simulink model "bins_model"  (Simulink 7.9)
settings: Solver=ode23  StartTime=0.0  StopTime=12  MaxStep=0.01  RelTol=1e-6
settings Model: Creator=S  LastModifiedBy=S
settings SolverCC: SolverResetMethod=Robust
settings CodeAppCC: CustomSymbolStrType=$N$R$M_T
settings GRTTargetCC: CodeReplacementLibrary=None  CPPClassGenCompliant=on

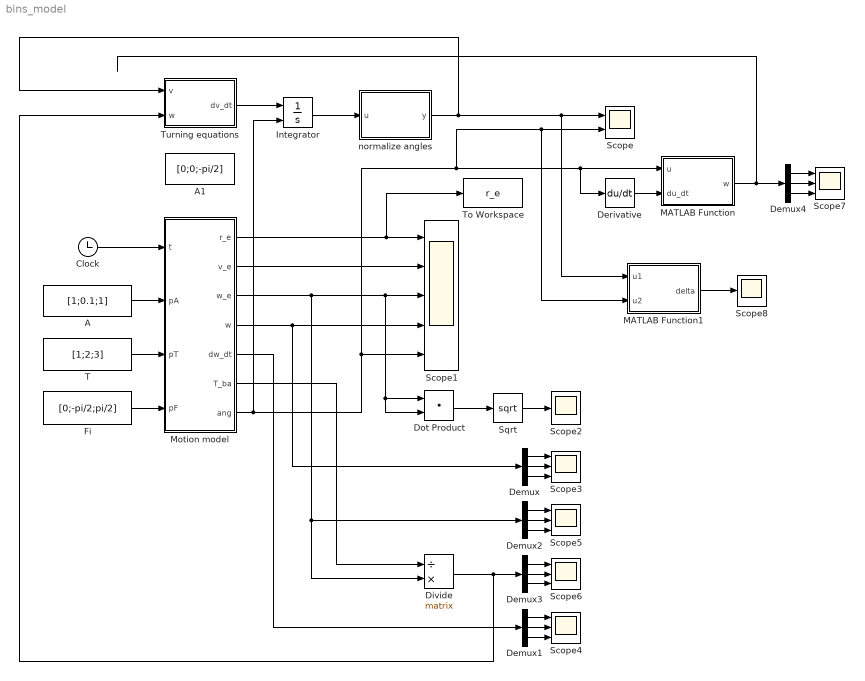
== system bins_model ==
  A : Constant  Value=[1;0.1;1]
  A1 : Constant  Value=[0;0;-pi/2]
  Clock : Clock
  Demux{,1..4} (5 alike) : Demux  Outputs=3
  Derivative : Derivative
  Divide : Product  Inputs=/*  Multiplication=Matrix(*)
  Dot Product : DotProduct  InputSameDT=on  OutDataTypeStr=Inherit: Inherit via internal rule
  Fi : Constant  Value=[0;-pi/2;pi/2]
  Integrator : Integrator  InitialConditionSource=external
  MATLAB Function : MATLAB Function  TreatAsAtomicUnit=on
  MATLAB Function1 : MATLAB Function  TreatAsAtomicUnit=on
  Motion model : MATLAB Function  TreatAsAtomicUnit=on
  Scope : Scope  NumInputPorts=2
      settings: TimeRange=3  YMin=-4~-4  YMax=4~4  MaxDataPoints=50000
  Scope1 : Scope  NumInputPorts=5
      settings: TimeRange=3  YMin=-1~-10~-20~-50~-5  YMax=1~10~40~50~5  MaxDataPoints=50000
  Scope2 : Scope
      settings: SaveName=ScopeData2  MaxDataPoints=50000
  Scope{3..7} (5 alike) : Scope  NumInputPorts=3
      Scope3 settings: TimeRange=1  YMin=-8~-2e-15~0  YMax=8~4e-15~10  SaveName=ScopeData3  MaxDataPoints=50000
      Scope4 settings: TimeRange=1  YMin=-2e-12~-20~-10  YMax=2e-12~20~10  SaveName=ScopeData4  MaxDataPoints=50000
      Scope5 settings: TimeRange=1  YMin=-30~-30~-8  YMax=30~30~8  SaveName=ScopeData5  MaxDataPoints=50000
      Scope6 settings: TimeRange=3  YMin=-10~-1~0  YMax=150~1~40  SaveName=ScopeData6  MaxDataPoints=50000
      Scope7 settings: TimeRange=3  YMin=-10~-1~0  YMax=150~1~40  SaveName=ScopeData7  MaxDataPoints=50000
  Scope8 : Scope
      settings: SaveName=ScopeData8
  Sqrt : Sqrt  SaturateOnIntegerOverflow=on
  T : Constant  Value=[1;2;3]
  To Workspace : ToWorkspace  VariableName=r_e  SampleTime=-1  SaveFormat=Timeseries
  Turning equations : MATLAB Function  TreatAsAtomicUnit=on
  normalize angles : MATLAB Function  TreatAsAtomicUnit=on
  wires:
  Turning equations/1(dv_dt) -> Integrator/1
  Clock/1 -> Motion model/1(t)
  Motion model/1(r_e) -> To Workspace/1, Scope1/1
  A/1 -> Motion model/2(pA)
  T/1 -> Motion model/3(pT)
  Fi/1 -> Motion model/4(pF)
  Motion model/4(w) -> Scope1/4, Demux/1
  Motion model/2(v_e) -> Scope1/2
  Motion model/7(ang) -> Scope1/5, MATLAB Function/1(u), Derivative/1, Scope/2, MATLAB Function1/2(u2), Integrator/2
  Dot Product/1 -> Sqrt/1
  Sqrt/1 -> Scope2/1
  Demux/1 -> Scope3/1
  Demux/2 -> Scope3/2
  Demux/3 -> Scope3/3
  Motion model/5(dw_dt) -> Demux1/1
  Demux1/1 -> Scope4/1
  Demux1/2 -> Scope4/2
  Demux1/3 -> Scope4/3
  normalize angles/1(y) -> Turning equations/1(v), Scope/1, MATLAB Function1/1(u1)
  Integrator/1 -> normalize angles/1(u)
  Motion model/3(w_e) -> Scope1/3, Dot Product/1, Dot Product/2, Demux2/1, Divide/2
  Demux2/1 -> Scope5/1
  Demux2/2 -> Scope5/2
  Demux2/3 -> Scope5/3
  Motion model/6(T_ba) -> Divide/1
  Demux3/2 -> Scope6/2
  Demux3/3 -> Scope6/3
  Demux3/1 -> Scope6/1
  Divide/1 -> Demux3/1, Turning equations/2(w)
  Derivative/1 -> MATLAB Function/2(du_dt)
  Demux4/2 -> Scope7/2
  Demux4/1 -> Scope7/1
  Demux4/3 -> Scope7/3
  MATLAB Function/1(w) -> Demux4/1
  MATLAB Function1/1(delta) -> Scope8/1

== matlab function Motion model ==
  data: t input double; r_e output double; pA input double; pT input double; pF input double; v_e output double; w_e output double; w output double; dw_dt output double; T_ba output double; ang output double
function [r_e, v_e, w_e, w, dw_dt, T_ba, ang] = fcn(t, pA, pT, pF)
%#codegen

    [r_e, v_e, w_e, dw_dt, T_ba, ang] = f_motion_model(t, pA, pT, pF);
    w = T_ba'*w_e;
%     w = w_e;

%     w(1) = 0;
%     w(2) = 0;

end

== matlab function Turning equations ==
  data: v input double; dv_dt output double; w input double
function dv_dt = fcn(v, w)
%#codegen

    dv_dt = f_turning_by_Euler(v, w);
    
end

== matlab function normalize angles ==
  data: u input double; y output double
function y = fcn(u)
%#codegen
y = u;
for i=1:length(y)
    y(i)=f_normalize_angle(u(i));
end

== matlab function MATLAB Function ==
  data: u input double; w output double; du_dt input double
function w = fcn(u, du_dt)
%#codegen

w = [0, sin(u(1)), 1;...
     sin(u(3)), cos(u(3))*cos(u(1)), 0;...
     cos(u(3)), -sin(u(3))*cos(u(1)), 0]*du_dt;

end

== matlab function MATLAB Function1 ==
  data: u1 input double; delta output double; u2 input double
function delta = fcn(u1, u2)
%#codegen

delta = f_angles_diff(u1,u2);

end
